simulink model "NearSpace_CMG_AttitudeValidation_SurfaceOnly_S05_yaw30"  (R2024a)
settings: Solver=ode4  StartTime=0.0  StopTime=60  FixedStep=.001  RelTol=1e-3
InitFcn:
  | init_paths;
model workspace (MAT data in the model file):
  disturbance_schedule = [0 0.2 0.4 0.6 0.8 1 1.2 1.4 1.6 1.8 2 2.2 ... (1204 elements, 301x4)]
  native_controller_template : object (value not decoded)
  native_reference_bank : object (value not decoded)
  reference_attitude_deg = [0 0.2 0.4 0.6 0.8 1 1.2 1.4 1.6 1.8 2 2.2 ... (1204 elements, 301x4)]
  reference_body_rate = [0 0.2 0.4 0.6 0.8 1 1.2 1.4 1.6 1.8 2 2.2 ... (1204 elements, 301x4)]
  reference_torque_nom = [0 0.2 0.4 0.6 0.8 1 1.2 1.4 1.6 1.8 2 2.2 ... (1204 elements, 301x4)]
  reference_window = [-1e-06 0.199999 0.399999 0.599999 0.799999 0.999999 1.199999 1.399999 1.599999 1.799999 1.999999 2.199999 ... (130032 elements, 301x432)]
libraries: aerolibprivatev1p5 x1
(part 2 of 2)

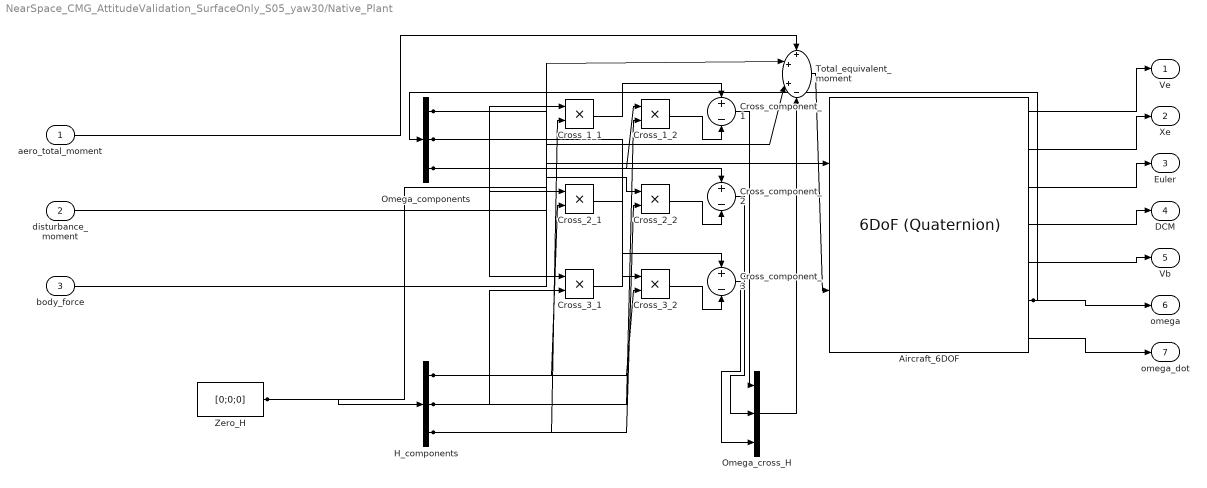
== system NearSpace_CMG_AttitudeValidation_SurfaceOnly_S05_yaw30/Native_Plant ==
  aero_total_moment : Inport  PortDimensions=3
  disturbance_moment : Inport  Port=2  PortDimensions=3
  body_force : Inport  Port=3  PortDimensions=3
  Aircraft_6DOF : aerolibprivatev1p5/6DoF (Quaternion)  xme_0=[0 0 0]  Vm_0=[0 0 0]  eul_0=[-1.7740922954857791e-18;0.21106173041320209;0.087266462599716474]  pm_0=[0 -0.0043273206504133811 -6.9388939039072284e-15]  Mass=1200  Inertia=[1200 0 0;0 8500 0;0 0 9000]  k_quat=1.0
  Cross_1_1 : Product
  Cross_1_2 : Product
  Cross_2_1 : Product
  Cross_2_2 : Product
  Cross_3_1 : Product
  Cross_3_2 : Product
  Cross_component_1 : Sum  Inputs=+-
  Cross_component_2 : Sum  Inputs=+-
  Cross_component_3 : Sum  Inputs=+-
  H_components : Demux  Outputs=3
  Omega_components : Demux  Outputs=3
  Omega_cross_H : Mux  Inputs=3
  Total_equivalent_moment : Sum  Inputs=+++-
  Zero_H : Constant  Value=[0;0;0]
  Ve : Outport
  Xe : Outport  Port=2
  Euler : Outport  Port=3
  DCM : Outport  Port=4
  Vb : Outport  Port=5
  omega : Outport  Port=6
  omega_dot : Outport  Port=7
  wires:
  Aircraft_6DOF/6 -> omega/1, Omega_components/1
  Zero_H/1 -> Total_equivalent_moment/3, H_components/1
  Omega_components/2 -> Cross_3_2/1, Cross_1_1/1
  H_components/3 -> Cross_2_2/2, Cross_1_1/2
  Omega_components/3 -> Cross_2_1/1, Cross_1_2/1
  H_components/2 -> Cross_3_1/2, Cross_1_2/2
  Cross_1_1/1 -> Cross_component_1/1
  Cross_1_2/1 -> Cross_component_1/2
  H_components/1 -> Cross_3_2/2, Cross_2_1/2
  Omega_components/1 -> Cross_3_1/1, Cross_2_2/1
  Cross_2_1/1 -> Cross_component_2/1
  Cross_2_2/1 -> Cross_component_2/2
  Cross_3_1/1 -> Cross_component_3/1
  Cross_3_2/1 -> Cross_component_3/2
  Cross_component_1/1 -> Omega_cross_H/1
  Cross_component_2/1 -> Omega_cross_H/2
  Cross_component_3/1 -> Omega_cross_H/3
  aero_total_moment/1 -> Total_equivalent_moment/1
  disturbance_moment/1 -> Total_equivalent_moment/2
  Omega_cross_H/1 -> Total_equivalent_moment/4
  Total_equivalent_moment/1 -> Aircraft_6DOF/2
  body_force/1 -> Aircraft_6DOF/1
  Aircraft_6DOF/1 -> Ve/1
  Aircraft_6DOF/2 -> Xe/1
  Aircraft_6DOF/3 -> Euler/1
  Aircraft_6DOF/4 -> DCM/1
  Aircraft_6DOF/5 -> Vb/1
  Aircraft_6DOF/7 -> omega_dot/1

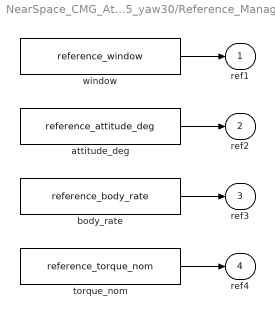
== system NearSpace_CMG_AttitudeValidation_SurfaceOnly_S05_yaw30/Reference_Manager ==
  attitude_deg : FromWorkspace  VariableName=reference_attitude_deg  Interpolate=off  OutputAfterFinalValue=Holding final value
  body_rate : FromWorkspace  VariableName=reference_body_rate  Interpolate=off  OutputAfterFinalValue=Holding final value
  torque_nom : FromWorkspace  VariableName=reference_torque_nom  Interpolate=off  OutputAfterFinalValue=Holding final value
  window : FromWorkspace  VariableName=reference_window  Interpolate=off  OutputAfterFinalValue=Holding final value
  ref1 : Outport
  ref2 : Outport  Port=2
  ref3 : Outport  Port=3
  ref4 : Outport  Port=4
  wires:
  window/1 -> ref1/1
  attitude_deg/1 -> ref2/1
  body_rate/1 -> ref3/1
  torque_nom/1 -> ref4/1
